simulink model "tester"  (R2024a)
settings: Solver=VariableStepAuto  StartTime=0.0  StopTime=inf  RelTol=1e-3
undefined symbols (not defined in the file): dt, I_charge_max, I_max, Id_char, Imax, Ion, Iq_char, Ki_d, Ki_q, Kp_d, Kp_q, lambda, Ld, Lithium, Lq, p, Rs, Soc_max, V_batt, Vdc_nom, Vs_max
libraries: mcbcontrolslib x4, simulink x2, spsBatteryLib x1, spsPermanentMagnetSynchronousMachineLib x1, spsSeriesRLCBranchLib x1, spsThreePhaseFaultLib x1, spsUniversalBridgeLib x1, sps_lib x1
(part 1 of 2)
settings Model: Creator=hirah  LastModifiedBy=hirah

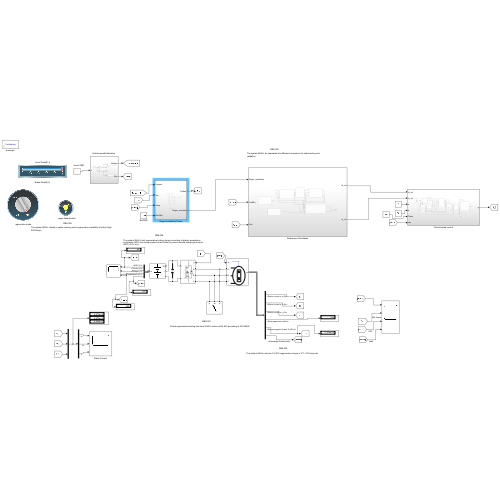
[thumbnail: Simulink's stored preview of the top-level diagram]
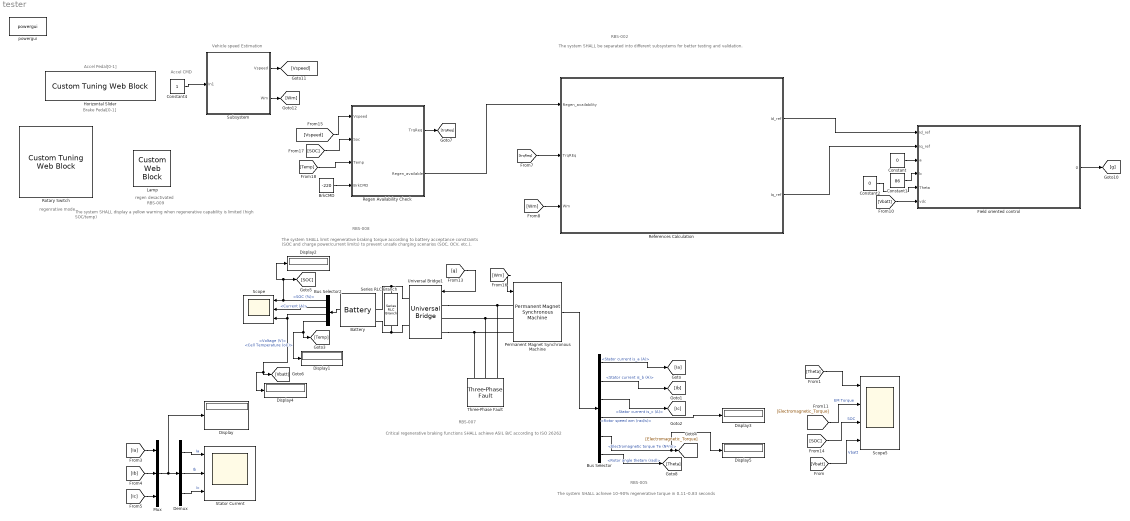
== system tester ==
  note: The system SHALL display a yellow warning when regenerative capability is limited (high SOC/temp)
  note: RBS-009
  note: RBS-008
  note: The system SHALL limit regenerative braking torque according to battery acceptance constraints (SOC and charge power/current limits) to prevent unsafe charging scenarios (SOC, OCV, etc.).
  note: RBS-007
  note: Critical regenerative braking functions SHALL achieve ASIL B/C according to ISO 26262
  note: RBS-005
  note: The system SHALL achieve 10–90% regenerative torque in 0.11–0.83 seconds
  note: RBS-002
  note: The system SHALL be separated into different subsystems for better testing and validation.
  note: regenrative mode
  note: regen desactivated
  note: Vehicle speed Estimation
  note: Accel CMD
  note: Accel Pedal[0-1]
  note: Brake Pedal[0-1]
  Battery : spsBatteryLib/Battery  BatType=Lithium-Ion  ShowTempParam=on  ThermalPreset=no  ShowAgeParam=off  NomV=750  NomQ=230  SOC=70  Batt_Tr=10  PresetModel=off  MaxQ=230  MinV=850  FullV=830  Dis_rate=100  R=0.030435  Normal_OP=208  expZone="[756.2701          11.3]"  current=[1.5 3]  Units=Ampere-hour  Tci=25  NomT=25  T2=-20  MaxQ2=173  FullV2=675  Normal_OP2=638  expZone2="[45           9]"  Rca=0.08  ti=3000  Dp=0  Neq0=0  Tsim=1e6  Ta1=25  Qeol=5.4*0.9  Reol=0.013333*1.2  Char_age=[2.3478, 3]  Dis_age=[2.3478, 10]  N1=1500  N2=10500  N3=1000  N4=1400  Ta2=45  N5=950
  BrkCMD : Constant  Value=-220
  Bus Selector : BusSelector  OutputSignals=Stator current is_a (A),Stator current is_b (A),Stator current is_c (A),Rotor speed wm (rad/s),Electromagnetic torque Te (N*m),Rotor angle thetam (rad)
  Bus Selector2 : BusSelector  OutputSignals=SOC (%),Current (A),Voltage (V),Cell Temperature (oC)
  Constant : Constant  Value=0
  Constant1 : Constant  Value=86
  Constant2 : Constant  Value=0
  Constant4 : Constant
  Demux : Demux  Outputs=3
  Display{,1..5} (6 alike) : Display
  Field oriented control : Subsystem
  Horizontal Slider : CustomTuningWebBlock  LabelPosition=Hide  ShowInitialText=on  Configuration="{\"components\":[{\"name\":\"LinearScaleComponent\",\"settings\":{\"bounds\":{\"max\":1,\"min\":0,\"tickInterval\":\"auto\"},\"internalTickHeightScaleFactor\":0.5,\"labelColor\":[255,255,200],\"labelFont\":{\"font\":\"Arial\",\"fontSize\":12},\"labelOffset\":0.05,\"labelTransparency\":1,\"needleImage\":{\"size\":[596,842],\"src\":\"data:image\\/svg+xml;base64,PD94bWwgdmVyc2lvbj0iMS4wIiBlbmNvZGluZz0idXRmLTgiPz4NCjwhLS0gR2VuZXJhdG9yOiBBZG9iZSBJbGx1c3RyYXRvciAyNS4wLjAsIFNWRyBFeHBvcnQgUGx1Zy1JbiAuIFNWRyBWZXJzaW9uOiA2LjAwIEJ1aWxkIDApICAtLT4NCjxzdmcgdmVyc2lvbj0iMS4xIg0KCSBpZD0ic3ZnOCIgeG1sbnM6Y2M9Imh0dHA6Ly9jcmVhdGl2ZWNvbW1vbnMub3JnL25zIyIgeG1sbnM6ZGM9Imh0dHA6Ly9wdXJsLm9yZy9kYy9lbGVtZW50cy8xLjEvIiB4bWxuczppbmtzY2FwZT0iaHR0cDovL3d3dy5pbmtzY2FwZS5vcmcvbmFtZXNw ...(+2420 chars)\",\"srcOrientation\":\"Right\"},\"needleOffset\":[-0.8044596912521441,-0.0642123287671233],\"needleSize\":{\"height\":0.4337797619047619,\"width\":0.07668067226890757},\"position\":[0.2829861111111111,0.04398634453781513,0.9196428571428571,0.6088789682539683],\"referencePoint\":\"auto\",\"scaleColors\":[],\"scaleColorsSize\":0.2,\"scaleDirection\":\"LR\",\"showLabels\":1,\"showMinorTicks\":0,\"showSpanLine\":1,\"showTicks\":1,\"tickColor\":[252,252,197],\"tickTransparency\":1,\"valueBarColor\":[0,114,189],\"valueBarOffset\":-0.27,\"valueBarSize\":0.1,\"valueBarTransparency\":1}},{\"name\":\"BackgroundImageComponent\",\"settings\":{\"image\":{\"size\":[380,101],\"src\":\"data:image\\/svg+xml;base64,PHN2ZyB4bWxucz0iaHR0cDovL3d3dy53My5vcmcvMjAwMC9zdmciIHhtbG5zOnhsaW5rPSJodHRwOi8vd3d3LnczLm9yZy8xOTk5L3hsaW5rIiB2aWV3Qm94PSIwIDAgMzgwIDEwMSI+PGRlZnM+PHN0eWxlPi5jbHMtMXtmaWxsOiMwMDJiNDI7fS5jbHMtMntmaWxsOiM0MjcwODI7fS5jbHMtM3tmaWxsOnVybCgjcmFkaWFsLWdyYWRpZW50KTt9LmNscy00e2ZpbGw6I2M4YzhjODtzdHJva2U6IzAwMDt9PC9zdHlsZT48cmFkaWFsR3JhZGllbnQgaWQ9InJhZGlhbC1ncmFkaWVudCIgY3g9IjE5MCIgY3k9IjUwLjUiIHI9IjI2OS4yMSIgZ3JhZGllbnRVbml0cz0idXNlclNwYWNlT25Vc2UiPjxzdG9wIG9mZnNldD0iMC4wMSIgc3RvcC1jb2xvcj0iIzNlNGY1OCIvPjxzdG9wIG9mZnNldD0iMC4wNiIgc3RvcC1jb2xvcj0iIzQ0NTc2MSIvPjxzdG9wIG9mZnNldD0iMC4xNSIgc3RvcC1jb2xvcj0iIzU1NmE3NiIvPjxzdG9wIG9mZnNldD0iMC4yNSIgc3RvcC1jb2xvcj0iIzZkODg5NSIvPjxzdG9wIG9mZnNldD0iMC4zOCIgc3RvcC1jb2xvcj0iIzhmYjJjMyIvPjxzdG9wIG9mZnNldD0iMC41MiIgc3RvcC1jb2xvcj0iI2I2ZTRmYSIvPjxzdG9wIG9mZnNldD0iMSIgc3RvcC1jb2xvcj0iIzE1NDY1NyIvPjwvcmFkaWFsR3JhZGllbnQ+PC9kZWZzPjxnIGlkPSJmcmFtZSI+PGcgaWQ9IkxheWVyXzIiIGRhdGEtbmFtZT0iTGF5ZXIgMiI+PGcgaWQ9IkxheWVyXzEtMiIgZGF0YS1uYW1lPSJMYXllciAxLTIiPjxyZWN0IGlkPSJyZWN0MTAzNiIgY2xhc3M9ImNscy0xIiB4PSIxMSIgeT0iMTEiIHdpZHRoPSIzNTgiIGhlaWdodD0iNzkiLz48cGF0aCBpZD0icGF0aDEwMzgiIGNsYXNzPSJjbHMtMiIgZD0iTTgsOFY5M0gzNzJWOFpNMzY5LDkwSDExVjExSDM2OVoiLz48cGF0aCBpZD0icGF0aDEwNDAiIGNsYXNzPSJjbHMtMyIgZD0iTTAsMFYxMDFIMzgwVjBaTTM3Miw5M0g4VjhIMzcyWiIvPjwvZz48L2c+PC9nPjxnIGlkPSJ0cmFjayI+PHBhdGggaWQ9InJlY3QxNjExIiBjbGFzcz0iY2xzLTQiIGQ9Ik0zMy4zNywyNi41OUgzNDYuNjNjNCwwLDcuMjUsMi42LDcuMjUsNS44MWgwYzAsMy4yMS0zLjI1LDUuODItNy4yNSw1LjgySDMzLjM3Yy00LDAtNy4yNS0yLjYxLTcuMjUtNS44MmgwQzI2LjEyLDI5LjE5LDI5LjM3LDI2LjU5LDMzLjM3LDI2LjU5WiIvPjwvZz48L3N2Zz4=\",\"srcOrientation\":\"horizontal\"},\"position\":[0,0,1,1],\"scaleMode\":\"0\"}},{\"name\":\"ForegroundImageComponent\",\"settings\":{\"image\":{\"size\":[0,0],\"src\":\"default\",\"srcOrientation\":[]},\"isForeground\":1,\"position\":[0,0,1,1],\"scaleMode\":\"0\"}}],\"settings\":{\"BindingType\":\"param\",\"aspectRatio\":3.7777777777777777,\"backgroundColor\":[0,0,0,\"1\"],\"backgroundOffset\":0,\"backgroundOpacity\":1,\"fixedAspectRatio\":\"on\",\"foregroundColor\":[252,252,196],\"orientation\":\"horizontal\",\"showBackgroundColor\":false,\"value\":0,\"version\":\"R2023a\"},\"type\":\"LinearGauge\"}"
  Lamp : CustomWebBlock  LabelPosition=Hide  ShowInitialText=on  Configuration="{\"components\":[{\"name\":\"BackgroundImageComponent\",\"settings\":{\"image\":{\"size\":[150,150],\"src\":\"data:image\\/svg+xml;base64,PHN2ZyB4bWxucz0iaHR0cDovL3d3dy53My5vcmcvMjAwMC9zdmciIHhtbG5zOnhsaW5rPSJodHRwOi8vd3d3LnczLm9yZy8xOTk5L3hsaW5rIiB2aWV3Qm94PSIwIDAgNTAwIDUwMCI+PGRlZnM+PHN0eWxlPi5he2ZpbGw6dXJsKCNhKTt9LmJ7ZmlsbDp1cmwoI2IpO30uY3tmaWxsOnVybCgjYyk7fTwvc3R5bGU+PHJhZGlhbEdyYWRpZW50IGlkPSJhIiBjeD0iMjgzLjg0IiBjeT0iLTQ2Ni4zNyIgcj0iMzc1Ljc1IiBncmFkaWVudFRyYW5zZm9ybT0ibWF0cml4KDEuMzksIDAsIDAsIC0xLjM5LCAtMTUzLjU2LCAtNjQ0LjA4KSIg ...(+2088 chars)\",\"srcOrientation\":\"Right\"},\"position\":[0,0,1,1],\"scaleMode\":\"0\"}},{\"name\":\"LampStateComponent\",\"settings\":{\"position\":[0,0,1,1],\"states\":[{\"icon\":{\"customSrc\":\"data:image\\/svg+xml;base64,PHN2ZyBpZD0iTGF5ZXJfMSIgZGF0YS1uYW1lPSJMYXllciAxIiB4bWxucz0iaHR0cDovL3d3dy53My5vcmcvMjAwMC9zdmciIHZpZXdCb3g9IjAgMCA0MTEgNDU4Ij48ZGVmcz48c3R5bGU+LmNscy0xe2ZpbGw6I2ZkZjhjMTt9LmNscy0ye2ZpbGw6I2ZlZTEwMDt9LmNscy0ze2ZpbGw6IzIzMWYyMDt9LmNscy00e2ZpbGw6I2EwOWY5Zjt9LmNscy00LC5jbHMtNSwuY2xzLTZ7c3Ryb2tlOiMyMzFmMjA7c3Ryb2tlLW1pdGVybGltaXQ6MTA7fS5jbHMtNXtmaWxsOiNmZmY7fS5jbHMtNntmaWxsOm5vbmU7fTwvc3R5bGU+PC9kZWZz ...(+5168 chars)\",\"id\":-1,\"srcOrientation\":\"Right\",\"type\":\"custom\"},\"iconScale\":0.8,\"metadata\":{},\"overlayType\":\"intersect\",\"shape\":{\"color\":[0.6509803921568628,0.6509803921568628,0.6509803921568628],\"opacity\":1,\"position\":[0.1,0.1,0.8,0.8],\"type\":\"ellipse\"},\"value\":[]},{\"icon\":{\"customSrc\":\"data:image\\/svg+xml;base64,PHN2ZyBpZD0iTGF5ZXJfMSIgZGF0YS1uYW1lPSJMYXllciAxIiB4bWxucz0iaHR0cDovL3d3dy53My5vcmcvMjAwMC9zdmciIHZpZXdCb3g9IjAgMCA0MTEgNDU4Ij48ZGVmcz48c3R5bGU+LmNscy0xe2ZpbGw6I2ZkZjhjMTt9LmNscy0ye2ZpbGw6I2ZlZTEwMDt9LmNscy0ze2ZpbGw6IzIzMWYyMDt9LmNscy00e2ZpbGw6I2EwOWY5Zjt9LmNscy00LC5jbHMtNSwuY2xzLTZ7c3Ryb2tlOiMyMzFmMjA7c3Ryb2tlLW1pdGVybGltaXQ6MTA7fS5jbHMtNXtmaWxsOiNmZmY7fS5jbHMtNntmaWxsOm5vbmU7fTwvc3R5bGU+PC9kZWZz ...(+5168 chars)\",\"id\":-1,\"srcOrientation\":\"Right\",\"type\":\"custom\"},\"iconScale\":0.8,\"metadata\":{\"useDefaults\":{\"customIcon\":true,\"icon\":true,\"overlayType\":true,\"shape\":true,\"sizeAndPosition\":true}},\"overlayType\":\"intersect\",\"shape\":{\"color\":[1,1,0.06666666666666667],\"opacity\":1,\"position\":[0.1,0.1,0.8,0.8],\"type\":\"ellipse\"},\"value\":\"0\"},{\"icon\":{\"customSrc\":\"data:image\\/svg+xml;base64,PHN2ZyBpZD0iTGF5ZXJfMSIgZGF0YS1uYW1lPSJMYXllciAxIiB4bWxucz0iaHR0cDovL3d3dy53My5vcmcvMjAwMC9zdmciIHZpZXdCb3g9IjAgMCA0MTEgNDU4Ij48ZGVmcz48c3R5bGU+LmNscy0xe2ZpbGw6I2ZkZjhjMTt9LmNscy0ye2ZpbGw6I2ZlZTEwMDt9LmNscy0ze2ZpbGw6IzIzMWYyMDt9LmNscy00e2ZpbGw6I2EwOWY5Zjt9LmNscy00LC5jbHMtNSwuY2xzLTZ7c3Ryb2tlOiMyMzFmMjA7c3Ryb2tlLW1pdGVybGltaXQ6MTA7fS5jbHMtNXtmaWxsOiNmZmY7fS5jbHMtNntmaWxsOm5vbmU7fTwvc3R5bGU+PC9kZWZz ...(+5168 chars)\",\"id\":-1,\"srcOrientation\":\"Right\",\"type\":\"custom\"},\"iconScale\":0.8,\"metadata\":{\"useDefaults\":{\"customIcon\":true,\"icon\":true,\"overlayType\":true,\"shape\":true,\"sizeAndPosition\":true}},\"overlayType\":\"intersect\",\"shape\":{\"color\":[0.14901960784313725,0.14901960784313725,0.14901960784313725],\"opacity\":1,\"position\":[0.1,0.1,0.8,0.8],\"type\":\"ellipse\"},\"value\":\"1\"}],\"valueType\":\"discrete\"}},{\"name\":\"ForegroundImageComponent\",\"settings\":{\"image\":{\"size\":[150,150],\"src\":\"data:image\\/svg+xml;base64,PHN2ZyB4bWxucz0iaHR0cDovL3d3dy53My5vcmcvMjAwMC9zdmciIHhtbG5zOnhsaW5rPSJodHRwOi8vd3d3LnczLm9yZy8xOTk5L3hsaW5rIiB2aWV3Qm94PSIwIDAgNTAwIDUwMCI+PGRlZnM+PHN0eWxlPi5he2ZpbGw6dXJsKCNhKTt9PC9zdHlsZT48bGluZWFyR3JhZGllbnQgaWQ9ImEiIHgxPSIxNzMuMDUiIHkxPSItNjI3Ljc4IiB4Mj0iMTczLjA1IiB5Mj0iLTUyMi40MyIgZ3JhZGllbnRUcmFuc2Zvcm09Im1hdHJpeCgxLjI5LCAwLCAwLCAtMS4zMywgMjcuMTMsIC02MjguMzEpIiBncmFkaWVudFVuaXRzPSJ1c2VyU3BhY2VPblVzZSI+PHN0b3Agb2Zmc2V0PSIwIiBzdG9wLWNvbG9yPSIjZmZmIiBzdG9wLW9wYWNpdHk9IjAuMjUiLz48c3RvcCBvZmZzZXQ9IjEiIHN0b3AtY29sb3I9IiNmZmYiIHN0b3Atb3BhY2l0eT0iMCIvPjwvbGluZWFyR3JhZGllbnQ+PC9kZWZzPjxwYXRoIGNsYXNzPSJhIiBkPSJNNDI5LjMsMTkwLjY2QzQwMi40NSwxMTQuNTEsMzMyLjY3LDYwLjE3LDI1MC44NSw2MC4xN2MtODMuNDMsMC0xNTQuMjgsNTYuNDItMTc5Ljk1LDEzNSwxNS4zNCwzOSw4OC4xMSw3LDE3Ny4wNyw3QzM0MCwyMDIuMDgsNDE3LjI2LDIzNi40Niw0MjkuMywxOTAuNjZaIi8+PC9zdmc+\",\"srcOrientation\":\"Right\"},\"isForeground\":1,\"position\":[0,0,1,1],\"scaleMode\":\"0\"}}],\"settings\":{\"BindingType\":\"signal\",\"aspectRatio\":1.032258064516129,\"backgroundColor\":[0,0,0],\"backgroundOffset\":0.14,\"backgroundOpacity\":1,\"blockOrientation\":\"Right\",\"fixedAspectRatio\":\"on\",\"showBackgroundColor\":false,\"value\":0,\"version\":\"R2023a\"},\"type\":\"Lamp\"}"  StateValueType=Discrete  Icon=Custom
  Mux : Mux  Inputs=3
  Permanent Magnet Synchronous Machine : spsPermanentMagnetSynchronousMachineLib/Permanent Magnet Synchronous Machine  NbPhases=3  FluxDistribution=Sinusoidal  RotorType=Salient-pole  MechanicalLoad=Speed w  PresetModel=No  ShowDetailedParameters=on  MeasurementBus=off  Resistance=0.012  Inductance=0.0144e-3  dqInductances=[0.0004 0.0008]  La=0.00153  MachineConstant=Flux linkage established by magnets (V.s)  Flux=0.095  VoltageCst=68.9244  TorqueCst=0.57  Flat=120  Mechanical=[0.01 0.001 4]  PolePairs=4  InitialConditions=[1000,0,0,0]  InitialConditions5ph=[0 0 0 0 0 0]  RefAngle=90 degrees behind phase A axis (modified Park)  IterativeDiscreteModel=Trapezoidal non iterative  TsBlock=-1  TsPowergui=0
  References Calculation : Subsystem
  Regen Availability Check : Subsystem
  Rotary Switch : CustomTuningWebBlock  LabelPosition=Hide  ShowInitialText=on  Configuration="{\"components\":[{\"name\":\"RotarySwitchComponent\",\"settings\":{\"arcAngle\":300,\"arcAngleOffset\":120,\"handle\":{\"size\":[150,150],\"src\":\"data:image\\/svg+xml;base64,PHN2ZyBpZD0iTGF5ZXJfMSIgZGF0YS1uYW1lPSJMYXllciAxIiB4bWxucz0iaHR0cDovL3d3dy53My5vcmcvMjAwMC9zdmciIHhtbG5zOnhsaW5rPSJodHRwOi8vd3d3LnczLm9yZy8xOTk5L3hsaW5rIiB2aWV3Qm94PSIwIDAgMTIxIDEyMSI+PGRlZnM+PHN0eWxlPi5jbHMtMXtmaWxsOnVybCgjbGluZWFyLWdyYWRpZW50KTt9LmNscy0yLC5jbHMtM3tmaWxsOiNkMWQxZDE7fS5jbHMtM3tzdHJva2U6I2I3YjdiNztzdHJva2UtbWl0ZXJsaW1pdDoxMDtzdHJva2Utd2lkdGg6MC4yNXB4O30uY2xzLTR7ZmlsbDojZjMwMDAwO30uY2xzLTV7ZmlsbDojZjIxNzY3O308L3N0eWxlPjxsaW5lYXJHcmFkaWVudCBpZD0ibGluZWFyLWdyYWRpZW50IiB4MT0iNjAuNSIgeTE9IjEyMC41IiB4Mj0iNjAuNSIgeTI9IjAuNSIgZ3JhZGllbnRVbml0cz0idXNlclNwYWNlT25Vc2UiPjxzdG9wIG9mZnNldD0iMCIgc3RvcC1jb2xvcj0iI2QxZDFkMSIvPjxzdG9wIG9mZnNldD0iMC4xIiBzdG9wLWNvbG9yPSIjY2VjZWNlIi8+PHN0b3Agb2Zmc2V0PSIwLjE5IiBzdG9wLWNvbG9yPSIjYzNjM2MzIi8+PHN0b3Agb2Zmc2V0PSIwLjI4IiBzdG9wLWNvbG9yPSIjYjFiMWIxIi8+PHN0b3Agb2Zmc2V0PSIwLjM2IiBzdG9wLWNvbG9yPSIjOTg5ODk4Ii8+PHN0b3Agb2Zmc2V0PSIwLjQ0IiBzdG9wLWNvbG9yPSIjNzg3ODc4Ii8+PHN0b3Agb2Zmc2V0PSIwLjQ2IiBzdG9wLWNvbG9yPSIjNmI2YjZiIi8+PHN0b3Agb2Zmc2V0PSIwLjU0IiBzdG9wLWNvbG9yPSIjNmI2YjZiIi8+PHN0b3Agb2Zmc2V0PSIwLjU2IiBzdG9wLWNvbG9yPSIjNzY3Njc2Ii8+PHN0b3Agb2Zmc2V0PSIwLjY0IiBzdG9wLWNvbG9yPSIjOTc5Nzk3Ii8+PHN0b3Agb2Zmc2V0PSIwLjcyIiBzdG9wLWNvbG9yPSIjYjBiMGIwIi8+PHN0b3Agb2Zmc2V0PSIwLjgxIiBzdG9wLWNvbG9yPSIjYzNjM2MzIi8+PHN0b3Agb2Zmc2V0PSIwLjkiIHN0b3AtY29sb3I9IiNjZGNkY2QiLz48c3RvcCBvZmZzZXQ9IjEiIHN0b3AtY29sb3I9IiNkMWQxZDEiLz48L2xpbmVhckdyYWRpZW50PjwvZGVmcz48Y2lyY2xlIGNsYXNzPSJjbHMtMSIgY3g9IjYwLjUiIGN5PSI2MC41IiByPSI2MCIvPjxwYXRoIGNsYXNzPSJjbHMtMiIgZD0iTTYwLjUsMUE1OS41LDU5LjUsMCwxLDEsMSw2MC41LDU5LjU3LDU5LjU3LDAsMCwxLDYwLjUsMW0wLTFBNjAuNSw2MC41LDAsMSwwLDEyMSw2MC41LDYwLjUsNjAuNSwwLDAsMCw2MC41LDBaIi8+PHJlY3QgY2xhc3M9ImNscy0zIiB4PSIwLjUiIHk9IjUxLjUiIHdpZHRoPSIxMjAiIGhlaWdodD0iMTgiIHJ4PSIzLjA0Ii8+PHJlY3QgY2xhc3M9ImNscy00IiB4PSI1Ljc1IiB5PSI1OC43NSIgd2lkdGg9IjE2IiBoZWlnaHQ9IjMiLz48cGF0aCBjbGFzcz0iY2xzLTUiIGQ9Ik0yMS4yNSw1OS4yNXYyaC0xNXYtMmgxNW0xLTFoLTE3djRoMTd2LTRaIi8+PC9zdmc+\"},\"handleOffset\":[0,0],\"handleOrientation\":180,\"handlePosition\":[0,0,1,1],\"handleSize\":{\"height\":0.5,\"width\":0.5},\"labelRadius\":0.36,\"position\":[0,0,1,1],\"states\":[{\"Label\":{\"color\":[0,0,0,1],\"icon\":{\"size\":[0,0],\"src\":[],\"srcOrientation\":\"Right\"},\"iconPlacement\":\"left\",\"opacity\":1,\"position\":[0.7345552884615385,0.6796274038461538],\"show\":true,\"text\":{\"content\":\"Off\",\"font\":\"Helvetica\",\"fontSize\":24}},\"Value\":-50},{\"Label\":{\"color\":[0,0,0,1],\"icon\":{\"size\":[0,0],\"src\":[],\"srcOrientation\":\"Right\"},\"iconPlacement\":\"left\",\"opacity\":1,\"position\":[0.35757211538461536,0.7603966346153846],\"show\":true,\"text\":{\"content\":\"Low\",\"font\":\"Helvetica\",\"fontSize\":24}},\"Value\":-100},{\"Label\":{\"color\":[0,0,0,1],\"icon\":{\"size\":[0,0],\"src\":[],\"srcOrientation\":\"Right\"},\"iconPlacement\":\"left\",\"opacity\":1,\"position\":[0.09603365384615385,0.46033653846153844],\"show\":true,\"text\":{\"content\":\"Medium\",\"font\":\"Helvetica\",\"fontSize\":24}},\"Value\":-150},{\"Label\":{\"color\":[0,0,0,1],\"icon\":{\"size\":[0,0],\"src\":[],\"srcOrientation\":\"Right\"},\"iconPlacement\":\"left\",\"opacity\":1,\"position\":[0.36532451923076925,0.1180889423076923],\"show\":true,\"text\":{\"content\":\"High\",\"font\":\"Helvetica\",\"fontSize\":24}},\"Value\":-220}],\"tickRadius\":0.32}},{\"name\":\"BackgroundImageComponent\",\"settings\":{\"image\":{\"size\":[155,150],\"src\":\"data:image\\/svg+xml;base64,PD94bWwgdmVyc2lvbj0iMS4wIiBlbmNvZGluZz0idXRmLTgiPz4NCjwhLS0gR2VuZXJhdG9yOiBBZG9iZSBJbGx1c3RyYXRvciAyNS4wLjAsIFNWRyBFeHBvcnQgUGx1Zy1JbiAuIFNWRyBWZXJzaW9uOiA2LjAwIEJ1aWxkIDApICAtLT4NCjxzdmcgdmVyc2lvbj0iMS4xIg0KCSBpZD0iTGF5ZXJfMl8xXyIgeG1sbnM6Y2M9Imh0dHA6Ly9jcmVhdGl2ZWNvbW1vbnMub3JnL25zIyIgeG1sbnM6ZGM9Imh0dHA6Ly9wdXJsLm9yZy9kYy9lbGVtZW50cy8xLjEvIiB4bWxuczppbmtzY2FwZT0iaHR0cDovL3d3dy5pbmtzY2FwZS5vcmcv ...(+4184 chars)\",\"srcOrientation\":\"Right\"},\"position\":[0,0,1,1],\"scaleMode\":\"0\"}},{\"name\":\"ForegroundImageComponent\",\"settings\":{\"image\":{\"size\":[0,0],\"src\":\"default\",\"srcOrientation\":[]},\"isForeground\":1,\"position\":[0,0,1,1],\"scaleMode\":\"0\"}}],\"settings\":{\"BindingType\":\"param\",\"backgroundColor\":[0,0,255,\"1\"],\"backgroundOffset\":1,\"fixedAspectRatio\":\"on\",\"image\":{\"size\":[150,150],\"src\":\"data:image\\/svg+xml;base64,PD94bWwgdmVyc2lvbj0iMS4wIiBlbmNvZGluZz0iVVRGLTgiIHN0YW5kYWxvbmU9Im5vIj8+CjwhLS0gR2VuZXJhdG9yOiBBZG9iZSBJbGx1c3RyYXRvciAxOS4yLjEsIFNWRyBFeHBvcnQgUGx1Zy1JbiAuIFNWRyBWZXJzaW9uOiA2LjAwIEJ1aWxkIDApICAtLT4KCjxzdmcKICAgeG1sbnM6ZGM9Imh0dHA6Ly9wdXJsLm9yZy9kYy9lbGVtZW50cy8xLjEvIgogICB4bWxuczpjYz0iaHR0cDovL2NyZWF0aXZlY29tbW9ucy5vcmcvbnMjIgogICB4bWxuczpyZGY9Imh0dHA6Ly93d3cudzMub3JnLzE5OTkvMDIvMjItcmRmLXN5bnRh ...(+9660 chars)\"},\"showBackgroundColor\":false,\"variant\":\"rotarySwitch\",\"version\":\"R2023a\"},\"type\":\"RotarySwitch\"}"
  Scope : Scope  NumInputPorts=3
  Scope5 : Scope  NumInputPorts=4
  Series RLC Branch : spsSeriesRLCBranchLib/Series RLC Branch  LConnTagsString=__new0  RConnTagsString=__new0  BranchType=C  Resistance=1  Inductance=1e-3  SetiL0=off  InitialCurrent=0  Capacitance=75e-3  Setx0=off  InitialVoltage=0  Measurements=None
  Stator Current : Scope  NumInputPorts=3
  Subsystem : Subsystem
  Three-Phase Fault : spsThreePhaseFaultLib/Three-Phase Fault  InitialStates=0  FaultA=on  FaultB=on  FaultC=on  GroundFault=on  SwitchTimes="[1/60  5/60]"  External=off  SwitchStatus=NaN  FaultResistance=0.001  GroundResistance=0.01  SnubberResistance=1e6  SnubberCapacitance=inf  Measurements=None
  Universal Bridge1 : spsUniversalBridgeLib/Universal Bridge  Arms=3  SnubberResistance=1e5  SnubberCapacitance=inf  Device=MOSFET / Diodes  Ron=1e-3  Lon=0  ForwardVoltages="[  0  0  ]"  ForwardVoltage=0  GTOparameters=[ 10e-6 , 20e-6 ]  IGBTparameters=[ 1e-6 , 2e-6 ]  Measurements=None  Measurements_2=None  converterType=Rectifier
  powergui : sps_lib/powergui  Priority=1  SimulationMode=Continuous  SampleTime=50e-6  frequency=60  Iterations=50  frequencyindice=0  Pbase=100e6  ErrMax=1e-4  UnitsV=kV  UnitsW=MW  buscounter=0  FunctionMessages=off  echomessages=off  EnableUseOfTLC=off  CurrentSourceSwitches=off  DisableSnubberDevices=off  DisableRonSwitches=off  DisableVfSwitches=off  DisplayEquations=off  AutomaticDiscreteSolvers=off  SolverType=Tustin/Backward Euler (TBE)  Interpol=off  ExternalGateDelay=off  methode=off  Ts=100  x0status=blocks  SPID=on  SwTol=0  HookPort=off  NonlinearTolerance=1e-4  nMaxIteration=100  ContinueOnMaxIteration=off  RestoreLinks=warning  ResistiveCurrentMeasurement=off  Frange=[0:2:500]  Ylog=off  Xlog=on  ShowGrid=off  save=off  variable=ZData  structure=0  ZoomFFT=off  StartTime=0.0  cycles=1  DisplayStyle=1  fundamental=60  FreqAxis=off  MaxFrequency=1000  frequencyindicesteady=1  RmsSteady=1  display=off
  wires:
  [Vspeed] -> Regen Availability Check/1(Vspeed)
  Regen Availability Check/1(TrqReq) -> [trqReq]
  Bus Selector2/1 -> [SOC], Display2/1, Scope/1  "<SOC (%)>"
  Bus Selector2/2 -> Scope/2  "<Current (A)>"
  Battery/1 -> Bus Selector2/1
  Bus Selector2/3 -> Display4/1, [Vbatt], Scope/3  "<Voltage (V)>"
  [g] -> Universal Bridge1/1
  Bus Selector/3 -> [Ic]  "<Stator current is_c (A)>"
  Bus Selector/6 -> [Theta]  "<Rotor angle thetam (rad)>"
  Bus Selector/4 -> Display3/1  "<Rotor speed wm (rad/s)>"
  Bus Selector/1 -> [Ia]  "<Stator current is_a (A)>"
  Bus Selector/5 -> Display5/1, [Electromagnetic_Torque]  "<Electromagnetic torque Te (N*m)>"
  Bus Selector/2 -> [Ib]  "<Stator current is_b (A)>"
  Permanent Magnet Synchronous Machine/1 -> Bus Selector/1
  [Ib] -> Mux/2
  [SOC] -> Scope5/3  "SOC"
  Demux/2 -> Stator Current/2  "Ib"
  [Ia] -> Mux/1
  [Electromagnetic_Torque] -> Scope5/2  "EM Torque"
  [Ic] -> Mux/3
  Mux/1 -> Display/1, Demux/1
  Demux/1 -> Stator Current/1  "Ia"
  Demux/3 -> Stator Current/3  "Ic"
  [Theta] -> Scope5/1
  [Vbatt] -> Scope5/4  "Vbatt"
  [Vbatt] -> Field oriented control/6(vdc)
  Constant2/1 -> Field oriented control/5(Theta)
  Constant/1 -> Field oriented control/3(a)
  Field oriented control/1(g) -> [g]
  [Wm] -> Permanent Magnet Synchronous Machine/1
  Constant4/1 -> Subsystem/1(In1)
  Subsystem/1(Vspeed) -> [Vspeed]
  Subsystem/2(Wm) -> [Wm]
  Bus Selector2/4 -> Display1/1, [Temp]  "<Cell Temperature (oC)>"
  [SOC] -> Regen Availability Check/2(Soc)
  [Temp] -> Regen Availability Check/3(Temp)
  References Calculation/1(Id_ref) -> Field oriented control/1(Id_ref)
  References Calculation/2(Iq_ref) -> Field oriented control/2(Iq_ref)
  Regen Availability Check/2(Regen_available) -> References Calculation/1(Regen_availability)
  [trqReq] -> References Calculation/2(TrqREq)
  [Wm] -> References Calculation/3(Wm)
  BrkCMD/1 -> Regen Availability Check/4(BrkCMD)
  Constant1/1 -> Field oriented control/4(b)
  connections:
  Battery/LConn2 -- Universal Bridge1/RConn2 -- Series RLC Branch/RConn1
  Universal Bridge1/RConn1 -- Battery/LConn1 -- Series RLC Branch/LConn1
  Three-Phase Fault/LConn3 -- Permanent Magnet Synchronous Machine/LConn3 -- Universal Bridge1/LConn3
  Universal Bridge1/LConn2 -- Three-Phase Fault/LConn2 -- Permanent Magnet Synchronous Machine/LConn2
  Three-Phase Fault/LConn1 -- Permanent Magnet Synchronous Machine/LConn1 -- Universal Bridge1/LConn1
